simulink model "regulacja"  (R2026a)
settings: Solver=VariableStepAuto  MaxStep=1
values from neighbouring files (symbols this model uses):
  czas_skok = 500    [KociolBud_Badania.m]
  dSP = 1    [KociolBud_Badania.m]
  k = 8 / (0.2*QkN)    [KociolBud_Badania.m]
  Ki_mp = 1/Ti_mp    (= 0.0030303030303)    [KociolBud_Badania.m]
  Ki_st = 1/Ti_st    (= 0.00666666666667)    [KociolBud_Badania.m]
  Kp_mp = 0.9/a_mp    [KociolBud_Badania.m]
  Kp_st = 0.9/a_st    [KociolBud_Badania.m]
  SP0 = Twew0(1)    [KociolBud_Badania.m]
  T0_mp = t2 - T_mp    (= 110)    [KociolBud_Badania.m]
  T0_st = 50    [KociolBud_Badania.m]
  T_mp = 1.5*(t2 - t1)    (= 360)    [KociolBud_Badania.m]
  T_st = 500    [KociolBud_Badania.m]
undefined symbols (not defined in the file or in its folder): Twew0
settings Model: Creator=mmaks  LastModifiedBy=mmaks

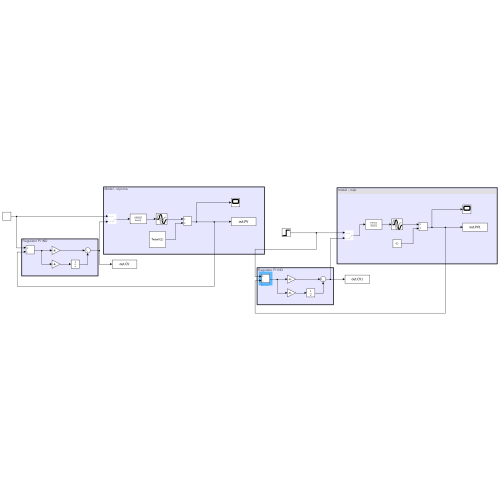
[thumbnail: Simulink's stored preview of the top-level diagram]
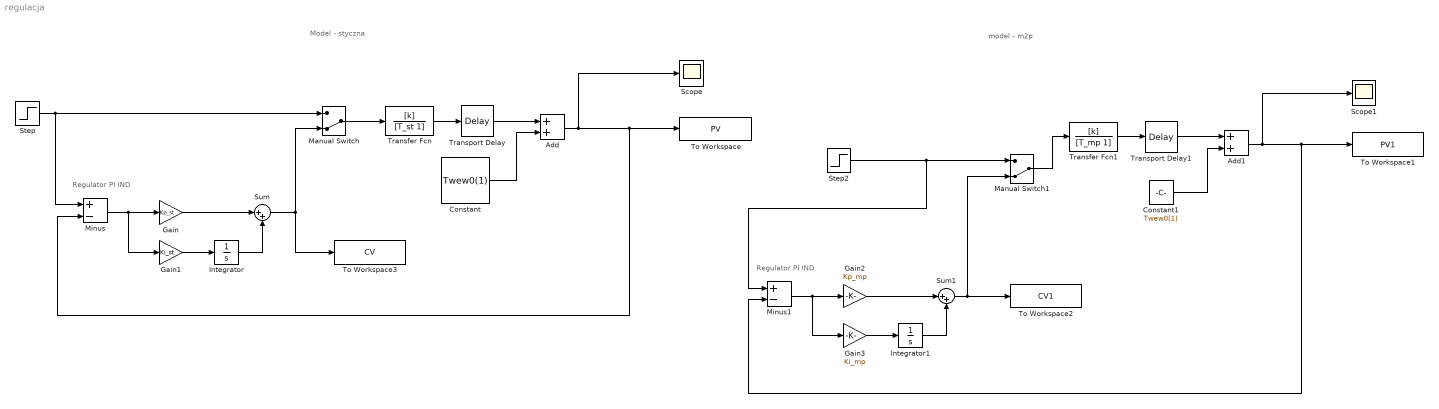
== system regulacja ==
  note: Regulator PI IND
  note: model - m2p
  note: Model - styczna
  note: Regulator PI IND
  Add : Sum
  Add1 : Sum
  Constant : Constant  Value=Twew0(1)
  Constant1 : Constant  Value=Twew0(1)
  Gain : Gain  Gain=Kp_st
  Gain1 : Gain  Gain=Ki_st
  Gain2 : Gain  Gain=Kp_mp
  Gain3 : Gain  Gain=Ki_mp
  Integrator : Integrator
  Integrator1 : Integrator
  Manual Switch : ManualSwitch  CurrentSetting=0
  Manual Switch1 : ManualSwitch  CurrentSetting=0
  Minus : Sum  Inputs=+-
  Minus1 : Sum  Inputs=+-
  Scope : Scope
      settings: ActiveDisplayYMinimum=11.000000000000025  ActiveDisplayYMaximum=31.000000000000025
  Scope1 : Scope
      settings: ActiveDisplayYMinimum=11.000000000000025  ActiveDisplayYMaximum=31.000000000000025
  Step : Step  Time=czas_skok  InitialValue=SP0  FinalValue=SP0 + dSP  SampleTime=0
  Step2 : Step  Time=czas_skok  InitialValue=SP0  FinalValue=SP0 + dSP  SampleTime=0
  Sum : Sum  Inputs=|++
  Sum1 : Sum  Inputs=|++
  To Workspace : ToWorkspace  VariableName=PV  SampleTime=-1
  To Workspace1 : ToWorkspace  VariableName=PV1  SampleTime=-1
  To Workspace2 : ToWorkspace  VariableName=CV1  SampleTime=-1
  To Workspace3 : ToWorkspace  VariableName=CV  SampleTime=-1
  Transfer Fcn : TransferFcn  Numerator=[k]  Denominator=[T_st 1]
  Transfer Fcn1 : TransferFcn  Numerator=[k]  Denominator=[T_mp 1]
  Transport Delay : TransportDelay  DelayTime=T0_st
  Transport Delay1 : TransportDelay  DelayTime=T0_mp
  wires:
  Transfer Fcn/1 -> Transport Delay/1
  Transport Delay/1 -> Add/1
  Step/1 -> Minus/1, Manual Switch/1
  Constant/1 -> Add/2
  Transfer Fcn1/1 -> Transport Delay1/1
  Transport Delay1/1 -> Add1/1
  Constant1/1 -> Add1/2
  Gain/1 -> Sum/1
  Integrator/1 -> Sum/2
  Gain1/1 -> Integrator/1
  Minus/1 -> Gain1/1, Gain/1
  Manual Switch/1 -> Transfer Fcn/1
  Sum/1 -> To Workspace3/1, Manual Switch/2
  Add/1 -> Scope/1, Minus/2, To Workspace/1
  Gain3/1 -> Integrator1/1
  Add1/1 -> Scope1/1, Minus1/2, To Workspace1/1
  Integrator1/1 -> Sum1/2
  Sum1/1 -> To Workspace2/1, Manual Switch1/2
  Gain2/1 -> Sum1/1
  Step2/1 -> Minus1/1, Manual Switch1/1
  Minus1/1 -> Gain3/1, Gain2/1
  Manual Switch1/1 -> Transfer Fcn1/1
